simulink model "aBaja2026"  (R2026a)
settings: Solver=FixedStepAuto  StartTime=0  StopTime=1000  FixedStep=timeStep
PostLoadFcn:
  | helperSLTrajectoryFollowerWithRRScenarioSetup
InitFcn:
  | helperSLTrajectoryFollowerWithRRScenarioSetup
  | worldActor=rrSim.getScenario();
  | world = worldActor.actor_spec.world_spec;
  | % Inputs you already have (example):
  | EgoActorID  = 1;
  | egoSetSpeed = 0;
  | 
  | % Get world + actors
  | 
  | 
  | % --- Find the ego actor (vectorized, minimal overhead) ---
  | actorIDs = arrayfun(@(a) str2double(a.actor_runtime.id), world.actors);
  | idx = (actorIDs == EgoActorID);
  | 
  | if nnz(idx) ~= 1
  |     error("Actor with ActorID:%d does not exist (or is not unique).", EgoActorID);
  | end
  | 
  | ego = world.actors(idx);
  | 
  | % --- Build 4x4 pose matrix quickly ---
  | temp_m = ego.actor_runtime.pose.matrix;
  | pose = [temp_m.col0.x temp_m.col1.x temp_m.col2.x temp_m.col3.x; ...
  |         temp_m.col0.y temp_m.col1.y temp_m.col2.y temp_m.col3.y; ...
  |         temp_m.col0.z temp_m.col1.z temp_m.col2.z temp_m.col3.z; ...
  |         temp_m.col0.w temp_m.col1.w temp_m.col2.w temp_m.col3.w];
  | 
  | rotm = pose(1:3,1:3);
  | pos  = pose(1:3,4)';   % [x y z] meters
  | 
  | % --- Euler angles from rotation matrix (ZYX: yaw, pitch, roll) ---
  | % If you have Robotics System Toolbox, rotm2eul exists; otherwise keep internal.
  | if exist("rotm2eul","file")
  |     eulZYX = rotm2eul(rotm,"ZYX");                 % radians: [yaw pitch roll]
  | else
  |     eulZYX = robotics.internal.rotm2eul(rotm,"ZYX");% radians: [yaw pitch roll]
  | end
  | 
  | % RoadRunner yaw -> conventional yaw:
  | yawDeg   = rad2deg(eulZYX(1)) + 90;
  | yawDeg   = mod(yawDeg + 180, 360) - 180;           % wrap to (-180,180]
  | pitchDeg = rad2deg(eulZYX(2));
  | rollDeg  = rad2deg(eulZYX(3));
  | 
  | % --- (Optional) reproduce your actorPose struct (kept consistent) ---
  | vGlobal = [egoSetSpeed*cosd(yawDeg), egoSetSpeed*sind(yawDeg), 0];
  | vBody   = (rotm' * vGlobal')';                      % body-fixed velocity
  | 
  | actorPose = struct( ...
  |     'ActorID', double(EgoActorID), ...
  |     'Position', pos, ...
  |     'Velocity', vGlobal, ...
  |     'vehicleFrameVelocity', [vBody(2), -vBody(1), vBody(3)], ...
  |     'Roll',  rollDeg, ...
  |     'Pitch', pitchDeg, ...
  |     'Yaw',   yawDeg, ...
  |     'AngularVelocity', [0 0 0]);
  | 
  | % --- Inline replacement for poseToSim3DInputs ---
  | % IMPORTANT: your original poseToSim3DInputs uses radians (pi terms),
  | % but getActorPose produced degrees. Fix by converting degrees -> radians here.
  | rollRad  = deg2rad(rollDeg);
  | pitchRad = deg2rad(pitchDeg);
  | yawRad   = deg2rad(yawDeg);
  | 
  | initialPosition = pos.*[1 -1 1];                               % 1x3
  | initialRotation = [rollRad, pitchRad, - yawRad];
  | 
  | % (Optional) wrap sim3D yaw to [-pi, pi]
  | initialRotation(3) = mod(initialRotation(3) + pi, 2*pi) - pi;
  | 
  | % Your original outputs:
  | % [initialPosition, initialRotation] = poseToSim3DInputs(...)
undefined symbols (not defined in the file): Defined, Ego, Lane, LKA, m, matlabshared, n, Pose, Sim3dSensor, timeStep, User, Velocity
libraries: roadrunnerscenario x9, drivingvehiclecontroller x3, simulink_extras x3, sim3dautolib x2, drivingscenarioandsensors x1, sim3dcameralib x1, sim3dlib x1, simulink x1
(part 1 of 2)
CloseFcn:
  | helperSLTrajectoryFollowerWithRRScenarioCleanup
settings Model: Creator=The MathWorks, Inc.  LastModifiedBy=rithv
settings DataIOCC: InspectSignalLogs=on
settings RTWCC: GenCodeOnly=on  GenerateReport=on  TargetLang=C++
settings GRTTargetCC: TargetLangStandard=C++03 (ISO)  CodeInterfacePackaging=C++ class

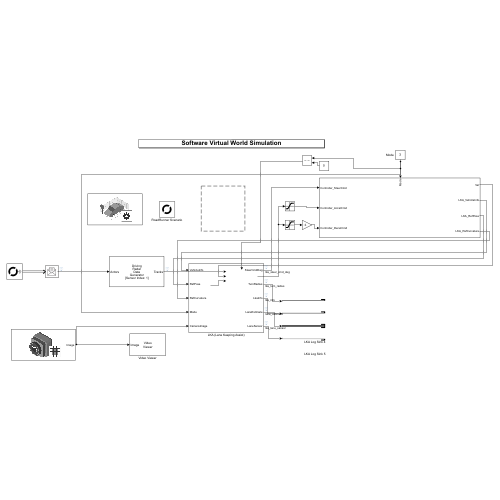
[thumbnail: Simulink's stored preview of the top-level diagram]
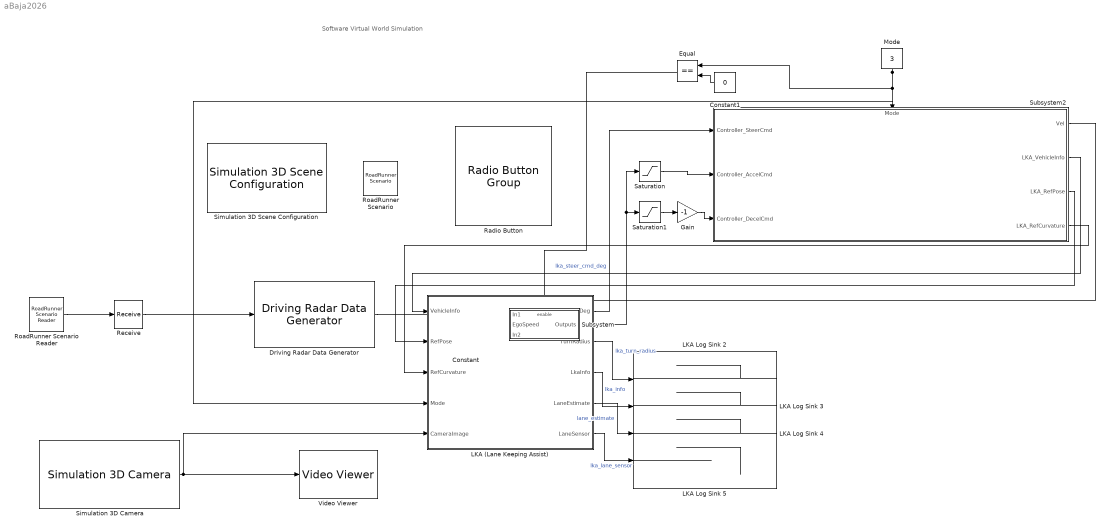
== system aBaja2026 ==
  note: Software Virtual World Simulation
  Constant : Constant  Value=8.3
  Constant1 : Constant  Value=0
  Driving Radar Data Generator : drivingscenarioandsensors/Driving Radar Data Generator  SensorIndex=1  UpdateRate=20  MountingLocation=[ 3.4, 0, 0.2 ]  MountingAngles=[0 0 0]  HasElevation=off  HasRangeRate=on  HasNoise=on  HasFalseAlarms=on  HasOcclusion=on  MaxNumReportsSource=Property  MaxNumReports=50  TargetReportFormat=Tracks  DetectionCoordinates=Body  TrackCoordinates=Body  BusNameSource=Auto  BusName=BusDrivingRadarDataGenerator  SimulateUsing=Interpreted execution  AzimuthResolution=4  ElevationResolution=5  RangeResolution=2.5  RangeRateResolution=0.5  AzimuthBiasFraction=0.1  ElevationBiasFraction=0.1  RangeBiasFraction=0.05  RangeRateBiasFraction=0.05  FieldOfView=[ 20, 5 ]  RangeLimits=[ 0, 150 ]  RangeRateLimits=[ -100, 100 ]  DetectionProbability=0.9  FalseAlarmRate=1e-06  ReferenceRange=100  ReferenceRCS=0  CenterFrequency=77e9  FilterInitializationFcn=initcvekf  ConfirmationThreshold=[2 3]  DeletionThreshold=[5 5]  InitialSeedSource=Repeatable  InitialSeed=0  UsedSeed=matlabshared.tracking.internal.SimulinkUtilities.seedManager(gcb)  ProfilesSource=From Scenario Reader block  ProfilesParameters=driving.internal.ActorProfilesRadarParameters  ProfilesExpression=struct('ClassID',0,'Length',4.7,'Width',1.8,'Height',1.4,'OriginOffset',[-1.35 0 0],'RCSPattern',[10 10;10 10],'RCSAzimuthAngles',[-180 180],'RCSElevationAngles',[-90 90])
  Equal : RelationalOperator  Operator===  OutDataTypeStr=boolean  RndMeth=Simplest  InputSameDT=off
  Gain : Gain  Gain=-1
  LKA (Lane Keeping Assist) : Subsystem  Description=aBaja 2026 LKA: lane source (camera detector YOLOP / team CNN / classic, or emulated for development), wheel-speed and gyro models, LKA_Controller (lane tracker, supervisor, pure pursuit / Stanley 2025 / MPC, a_y-jerk limiter, actuator manager). Output: road-wheel angle [deg, + left] to Subsystem2/Controller_SteerCmd.
  LKA Log Sink {2..5} (4 alike) : Terminator
  Mode : Constant  Value=3
  Radio Button : RadioButtonGroup  SelectedLabel=No Controller  ButtonGroupName=Event
  Receive : Receive  InputPortMessageModes=m  UseInternalQueue=off  QueueOverwriting=on  QueueLength=1  QueueType=LIFO
  RoadRunner Scenario : roadrunnerscenario/RoadRunner Scenario  ScenarioFileName=auto  ActorIDLinkedToModel=1  SampleTime=0.02  OpenRoadRunnerAtSimulationStart=on  EnableSimulationLoggingInRoadRunner=off  UserDefinedActions={}  UserDefinedEvents={}  PathPoints=500
  RoadRunner Scenario Reader : roadrunnerscenario/RoadRunner Scenario Reader  TopicCategory=Sensor  ActorCategory=All Types  ActionType=Path Following  EventType=User-Defined  TopicType=Actor Specifications  VehicleType=Vehicle Specifications  TrafficSignalType=Traffic Signal Specifications  TrafficSignalControllerType=Traffic Signal Controller Specifications  UserDefinedAction=Action1  UserDefinedEvent=Event1  Filter=Self  AdditionalRelationship=None  SensorTopic=Target Poses  LaneBoundaryOutputTopic=Ego-Lane  SensorID=1  SampleTime=0
  Saturation : Saturate  UpperLimit=2  LowerLimit=0
  Saturation1 : Saturate  UpperLimit=0  LowerLimit=-10
  Simulation 3D Camera : sim3dcameralib/Simulation 3D Camera  Priority=1  sensorTag=Sim3dSensor�  sensorId=1  sensorName=Sim3dSensor�  vehTagList={'Scene Origin';'SimulinkVehicle1';'SimulinkVehicle5'}  vehTag=SimulinkVehicle5  CoordinateSystem=ISO8855  mountLoc=Hood center  offsetFlag=off  tmountOffset=[0, 0, 0]  extTmount=off  rmountOffset=[0, 0, 0]  extRmount=off  FocalLength=[1109, 1109]  OpticalCenter=[640, 360]  ImageSize=[720, 1280]  RadialDistortion=[0, 0]  TangentialDistortion=[0, 0]  SensorSkew=0  VisualizeFieldOfView=on  FieldOfViewRange=61  DepthOutportEnabled=off  SemanticOutportEnabled=off  TransformOutportEnabled=off  SampleTime=-1  mountPoint=[0 0 0]  mountOrientation=[0 0 0]  aMode=3  ID=1
      settings: LibrarySourceBlock=drivingsim3d/Simulation 3D Camera
  Simulation 3D Scene Configuration : sim3dlib/Simulation 3D Scene Configuration  Priority=0  ProjectFormat=RoadRunner  SceneDesc=Straight road  ProjectName=D:\toolbox\shared\sim3d_projects\automotive_project_windows\UE\WindowsNoEditor\VehicleSimulation.exe  ScenePath=/Game/Maps/HwStrght  RoadRunnerProjectPath=D:\Work\25b\aBaja\SoftwareVirtualWorldSimulation\resources\UnrealFiles\AEB.usd  EnableOpenDRIVE=off  vehTagList={'Custom';'Scene Origin';'SimulinkVehicle1';'SimulinkVehicle5'}  vehTag=SimulinkVehicle5  AttachedCameraRelativeTranslation=[0 0 0]  FreeCameraDefaultInitialTranslation=[-6, 0, 2]  AttachedCameraRelativeRotation=[0 0 0]  FreeCameraDefaultInitialRotation=[0, -15, 0]  ViewpointName=Custom  FreeCameraInitialTranslation=[0 0 0]  FreeCameraInitialRotation=[0 0 0]  OpVisEn=off  Ts=timeStep  EnableWindow=off  EnableRemoteAccess=off  SimulationMode=CoSimulation  SimulateUsing=Interpreted execution  EnableAnimationRecording=off  OverrideDefaultRecording=off  AnimationRecordingFileName=sim3dAnimation.mat  AnimationRecordingInterval=[0 inf]  EnableWeather=off  SunAzimuth=90  SunAltitude=40.0  EnableGeospatialSun=off  Latitude=0  Longitude=0  Date=2023-01-01  Time=10:30:00  GeoTimeZone=-5.0  SunDaylightSaving=off  wind=1  clouds=10  EnableVolumetricClouds=off  CloudCoverage=0  CloudAltitude=6  fog=0  rain=0  RaindropsEffect=off  SnowDensity=0  EnableGeospatial=off  TilesetSource=Earth terrain  UseTrueOrigin=off  OriginHeight=200  OriginLatitude=40.744652  OriginLongitude=-73.988864  MapStyle=Aerial  AdditionalAssetIDs=[]  UseAdvancedSunSky=off  SolarTime=11  TimeZone=-5  Day=21  Month=9  Year=2022  UseDaylightSavingTime=on  DSTStartDay=10  DSTStartMonth=3  DSTEndDay=3  DSTEndMonth=11  DSTSwitchHour=2  sensorTag=MainCamera1  sensorId=1  sensorName=MainCamera1  mountLoc=Origin  offsetFlag=off  tmountOffset=[0, 0, 0]  rmountOffset=[0, 0, 0]  HorizontalResolution=1280  VerticalResolution=720  HorizontalFOV=60  mountPoint=[0 0 0]  mountOrientation=[0 0 0]  aMode=3  ID=1  GeoTrigger=Inactive  ViewNameList={'Custom'}  ViewTranslationList={'[0 0 0]'}  ViewRotationList={'[0 0 0]'}
      settings: LibrarySourceBlock=drivingsim3d/Simulation 3D Scene Configuration
  Subsystem : Subsystem
  Subsystem2 : Subsystem
      settings: PortSchema="{\"entries\":[{\"content\":{\"sides\":[{\"content\":{\"connectorIds\":[\"In1\",\"In2\",\"In3\"]},\"type\":\"ConnectorPlacement.EquallySpacedRectSide\",\"uuid\":\"2aff80b0-242f-49d2-ab36-0fd5582041a3\"},{\"content\":{\"connectorIds\":[\"Out1\",\"Out2\",\"Out3\",\"Out4\"],\"side\":\"RIGHT\"},\"type\":\"ConnectorPlacement.EquallySpacedRectSide\",\"uuid\":\"d3dd7aef-9728-4256-afed-548c516fba6e\"},{\"content\":{\"connectorIds\":[\"In4\"],\"side\":\"TOP\"},\"type\":\"ConnectorPlacement.EquallySpacedRectSide\",\"uuid\":\"fab05331-aabf-476e-ad1f-b5e3b7241bda\"}]},\"type\":\"ConnectorPlacement.EquallySpacedConnector\",\"uuid\":\"5fa4dbc3-4efd-4194-96c5-15d00eaf64f3\"}],\"packageUris\":[\"http://schema.mathworks.com/mf0/Connector/R2020b\"],\"version\":\"1.0\"}"
  Video Viewer : VideoViewer  FigPos=[1 1150 1920 1053]
  wires:
  RoadRunner Scenario Reader/1 -> Receive/1
  Receive/1 -> Driving Radar Data Generator/1
  Driving Radar Data Generator/1 -> Subsystem/1(In1)
  Subsystem2/1(Vel) -> Subsystem/2(EgoSpeed)
  Constant/1 -> Subsystem/3(In2)
  Subsystem/1(Outputs) -> Saturation/1, Saturation1/1
  Saturation/1 -> Subsystem2/2(Controller_AccelCmd)
  Saturation1/1 -> Gain/1
  Gain/1 -> Subsystem2/3(Controller_DecelCmd)
  Mode/1 -> Subsystem2/4(Mode), Equal/1, LKA (Lane Keeping Assist)/4(Mode)
  Equal/1 -> Subsystem/Enable
  Constant1/1 -> Equal/2
  Simulation 3D Camera/1 -> Video Viewer/1, LKA (Lane Keeping Assist)/5(CameraImage)
  Subsystem2/2(LKA_VehicleInfo) -> LKA (Lane Keeping Assist)/1(VehicleInfo)
  Subsystem2/3(LKA_RefPose) -> LKA (Lane Keeping Assist)/2(RefPose)
  Subsystem2/4(LKA_RefCurvature) -> LKA (Lane Keeping Assist)/3(RefCurvature)
  LKA (Lane Keeping Assist)/1(SteerCmdDeg) -> Subsystem2/1(Controller_SteerCmd)  "lka_steer_cmd_deg"
  LKA (Lane Keeping Assist)/2(TurnRadius) -> LKA Log Sink 2/1  "lka_turn_radius"
  LKA (Lane Keeping Assist)/3(LkaInfo) -> LKA Log Sink 3/1  "lka_info"
  LKA (Lane Keeping Assist)/4(LaneEstimate) -> LKA Log Sink 4/1  "lane_estimate"
  LKA (Lane Keeping Assist)/5(LaneSensor) -> LKA Log Sink 5/1  "lka_lane_sensor"

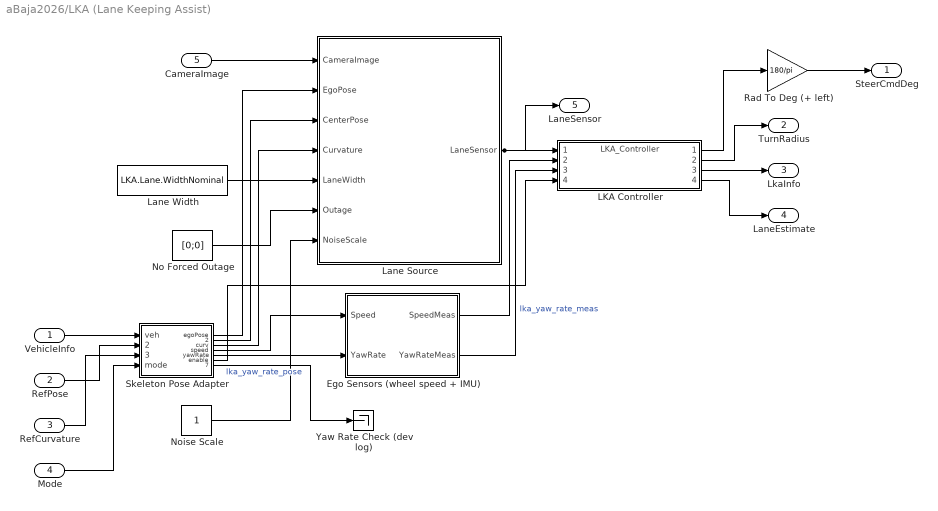
== system aBaja2026/LKA (Lane Keeping Assist) ==
  VehicleInfo : Inport
  RefPose : Inport  Port=2
  RefCurvature : Inport  Port=3
  Mode : Inport  Port=4
  CameraImage : Inport  Port=5
  Ego Sensors (wheel speed + IMU) : Subsystem
  LKA Controller : ModelReference  ModelNameDialog=LKA_Controller  SimulationMode=Normal  ModelReferenceVersion=1.1
  Lane Source : Subsystem  Variant=on
  Lane Width : Constant  Value=LKA.Lane.WidthNominal  SampleTime=LKA.Ts
  No Forced Outage : Constant  Value=[0;0]  SampleTime=LKA.Ts
  Noise Scale : Constant  SampleTime=LKA.Ts
  Rad To Deg (+ left) : Gain  Gain=180/pi
  Skeleton Pose Adapter : MATLAB Function  TreatAsAtomicUnit=on
  Yaw Rate Check (dev log) : Terminator
  SteerCmdDeg : Outport
  TurnRadius : Outport  Port=2
  LkaInfo : Outport  Port=3
  LaneEstimate : Outport  Port=4
  LaneSensor : Outport  Port=5
  wires:
  RefCurvature/1 -> Skeleton Pose Adapter/3(refCurv)
  VehicleInfo/1 -> Skeleton Pose Adapter/1(veh)
  No Forced Outage/1 -> Lane Source/6(Outage)
  LKA Controller/1 -> Rad To Deg (+ left)/1
  Lane Width/1 -> Lane Source/5(LaneWidth)
  RefPose/1 -> Skeleton Pose Adapter/2(refPose)
  Skeleton Pose Adapter/5(yawRate) -> Ego Sensors (wheel speed + IMU)/2(YawRate)
  Mode/1 -> Skeleton Pose Adapter/4(mode)
  CameraImage/1 -> Lane Source/1(CameraImage)
  Skeleton Pose Adapter/1(egoPose) -> Lane Source/2(EgoPose)
  Skeleton Pose Adapter/2(centerPose) -> Lane Source/3(CenterPose)
  Skeleton Pose Adapter/3(curv) -> Lane Source/4(Curvature)
  Skeleton Pose Adapter/4(speed) -> Ego Sensors (wheel speed + IMU)/1(Speed)
  LKA Controller/4 -> LaneEstimate/1
  Skeleton Pose Adapter/6(enable) -> LKA Controller/4
  Skeleton Pose Adapter/7(yawRatePose) -> Yaw Rate Check (dev log)/1  "lka_yaw_rate_pose"
  Ego Sensors (wheel speed + IMU)/1(SpeedMeas) -> LKA Controller/2
  Noise Scale/1 -> Lane Source/7(NoiseScale)
  Lane Source/1(LaneSensor) -> LaneSensor/1, LKA Controller/1
  Ego Sensors (wheel speed + IMU)/2(YawRateMeas) -> LKA Controller/3  "lka_yaw_rate_meas"
  LKA Controller/3 -> LkaInfo/1
  LKA Controller/2 -> TurnRadius/1
  Rad To Deg (+ left)/1 -> SteerCmdDeg/1

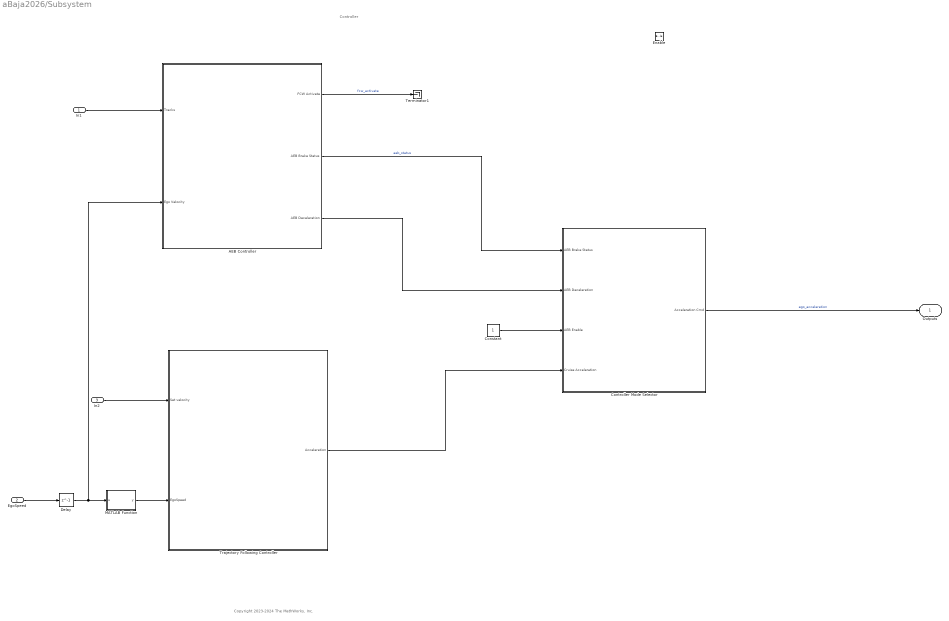
== system aBaja2026/Subsystem ==
  note: Controller
  note: Copyright 2023-2024 The MathWorks, Inc.
  In1 : Inport
  EgoSpeed : Inport  Port=2
  In2 : Inport  Port=3
  Enable : EnablePort
  AEB Controller : Subsystem
  Constant : Constant
  Controller Mode Selector : Subsystem
  Delay : Delay  DelayLength=1  InitialCondition=[0 0 0]
  MATLAB Function : MATLAB Function  TreatAsAtomicUnit=on
  Terminator1 : Terminator
  Trajectory Following Controller : Subsystem
  Outputs : Outport
  wires:
  Trajectory Following Controller/1(Acceleration) -> Controller Mode Selector/4(Cruise Acceleration)
  Delay/1 -> MATLAB Function/1(u), AEB Controller/2(Ego Velocity)
  In2/1 -> Trajectory Following Controller/1(Set velocity)
  MATLAB Function/1(y) -> Trajectory Following Controller/2(EgoSpeed)
  Controller Mode Selector/1(Acceleration Cmd) -> Outputs/1  "ego_acceleration"
  In1/1 -> AEB Controller/1(Tracks)
  AEB Controller/2(AEB Brake Status) -> Controller Mode Selector/1(AEB Brake Status)  "aeb_status"
  EgoSpeed/1 -> Delay/1
  Constant/1 -> Controller Mode Selector/3(AEB Enable)
  AEB Controller/1(FCW Activate) -> Terminator1/1  "fcw_activate"
  AEB Controller/3(AEB Deceleration) -> Controller Mode Selector/2(AEB Deceleration)

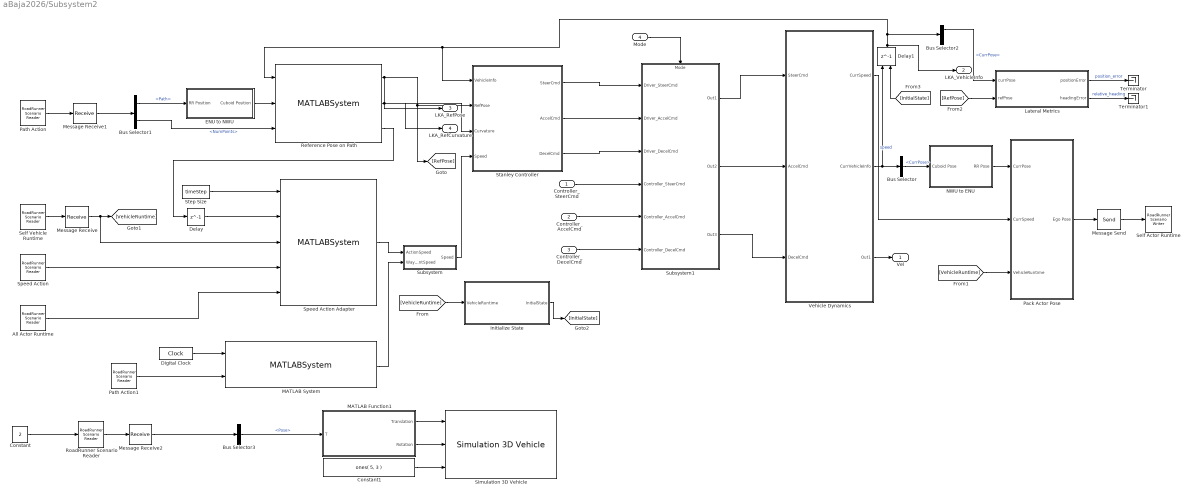
== system aBaja2026/Subsystem2 ==
  Controller_SteerCmd : Inport
  Controller_AccelCmd : Inport  Port=2
  Controller_DecelCmd : Inport  Port=3
  Mode : Inport  Port=4
  All Actor Runtime : roadrunnerscenario/RoadRunner Scenario Reader  TopicCategory=Actor  ActorCategory=All Types  ActionType=Path Following  EventType=User-Defined  TopicType=Actor Pose  VehicleType=Vehicle Specifications  TrafficSignalType=Traffic Signal Specifications  TrafficSignalControllerType=Traffic Signal Controller Specifications  UserDefinedAction=Action1  UserDefinedEvent=Event1  Filter=None  AdditionalRelationship=None  SensorTopic=Target Poses  LaneBoundaryOutputTopic=Ego-Lane  SensorID=1  SampleTime=0
  Bus Selector : BusSelector  OutputSignals=CurrPose
  Bus Selector1 : BusSelector  OutputSignals=PathTarget.Path,PathTarget.NumPoints
  Bus Selector2 : BusSelector  OutputSignals=CurrPose,CurrVelocity
  Bus Selector3 : BusSelector  OutputSignals=ActorRuntime.Pose
  Constant : Constant  Value=2  OutDataTypeStr=uint64
  Constant1 : Constant  Value=ones( 5, 3 )
  Delay : Delay  DelayLength=1  InitialCondition=logical(0)
  Delay1 : Delay  DelayLength=1  InitialConditionSource=Input port
      settings: InputPortMap=u0,p4
  Digital Clock : DigitalClock  SampleTime=-1
  ENU to NWU : Subsystem
  Initialize State : Subsystem
  Lateral Metrics : MATLAB Function  TreatAsAtomicUnit=on
  MATLAB Function1 : MATLAB Function  TreatAsAtomicUnit=on
  MATLAB System : MATLABSystem  InputPortMessageModes=n,m  System=getEgoSpeed  MaxNumPoints=5000
      mask Type: getEgoSpeed
  Message Receive : Receive  InputPortMessageModes=m
  Message Receive1 : Receive  InputPortMessageModes=m
  Message Receive2 : Receive  InputPortMessageModes=m
  Message Send : Send  OutputPortMessageModes=m
  NWU to ENU : Subsystem
  Pack Actor Pose : Subsystem
  Path Action : roadrunnerscenario/RoadRunner Scenario Reader  TopicCategory=Action  ActorCategory=All Types  ActionType=Path Following  EventType=User-Defined  TopicType=Actor Specifications  VehicleType=Vehicle Specifications  TrafficSignalType=Traffic Signal Specifications  TrafficSignalControllerType=Traffic Signal Controller Specifications  UserDefinedAction=Action1  UserDefinedEvent=Event1  Filter=Self  AdditionalRelationship=None  SensorTopic=Target Poses  LaneBoundaryOutputTopic=Ego-Lane  SensorID=1  SampleTime=0
  Path Action1 : roadrunnerscenario/RoadRunner Scenario Reader  TopicCategory=Action  ActorCategory=All Types  ActionType=Path Following  EventType=User-Defined  TopicType=Actor Specifications  VehicleType=Vehicle Specifications  TrafficSignalType=Traffic Signal Specifications  TrafficSignalControllerType=Traffic Signal Controller Specifications  UserDefinedAction=Action1  UserDefinedEvent=Event1  Filter=Self  AdditionalRelationship=None  SensorTopic=Target Poses  LaneBoundaryOutputTopic=Ego-Lane  SensorID=1  SampleTime=0
  Reference Pose on Path : MATLABSystem  System=HelperReferencePoseOnPath
      mask Type: HelperReferencePoseOnPath
  RoadRunner Scenario Reader : roadrunnerscenario/RoadRunner Scenario Reader  TopicCategory=Actor  ActorCategory=Vehicle  ActionType=Path Following  EventType=User-Defined  TopicType=Actor Specifications  VehicleType=Vehicle Pose  TrafficSignalType=Traffic Signal Specifications  TrafficSignalControllerType=Traffic Signal Controller Specifications  UserDefinedAction=Action1  UserDefinedEvent=Event1  Filter=Actor ID (provided by input)  AdditionalRelationship=None  SensorTopic=Target Poses  LaneBoundaryOutputTopic=Ego-Lane  SensorID=1  SampleTime=0
  Self Actor Runtime : roadrunnerscenario/RoadRunner Scenario Writer  TopicCategory=Actor  ActorCategory=All Types  EventType=Action Complete  UserDefinedEvent=Event1  VehicleType=Vehicle Pose  TopicType=Actor Pose
  Self Vehicle Runtime : roadrunnerscenario/RoadRunner Scenario Reader  TopicCategory=Actor  ActorCategory=Vehicle  ActionType=Path Following  EventType=User-Defined  TopicType=Actor Specifications  VehicleType=Vehicle Pose  TrafficSignalType=Traffic Signal Specifications  TrafficSignalControllerType=Traffic Signal Controller Specifications  UserDefinedAction=Action1  UserDefinedEvent=Event1  Filter=Self  AdditionalRelationship=None  SensorTopic=Target Poses  LaneBoundaryOutputTopic=Ego-Lane  SensorID=1  SampleTime=0
  Simulation 3D Vehicle : sim3dautolib/Simulation 3D Vehicle  Priority=-1  PassVehMesh=Muscle car  MeshPath=/MathWorksAutomotiveContent/Vehicles/Muscle/Meshes/SK_MuscleCar.SK_MuscleCar  VehColor=Black  ActorName=SimulinkVehicle1  VehLightsControl=off  HeadlightColor=[ 1, 1, 1 ]  HighBeamIntensity=100000  LowBeamIntensity=60000  HighBeamConeAngle=1.22  LowBeamConeAngle=1.22  LeftHeadlightOrientation=[ 0, 0 ]  RightHeadlightOrientation=[ 0, 0 ]  BrakelightIntensity=500  ReverselightIntensity=500  SignallightIntensity=500  SignallightPeriod=1  SignalPulseWidth=50  Translation=zeros( 5, 3 )  Rotation=zeros( 5, 3 )  Scale=ones( 5, 3 )  SampleTime=-1  ActorType=SimulinkVehicle  ID=1  aMode=2  ActorTag=SimulinkVehicle1
      settings: LibrarySourceBlock=vehdynlibsim3d/Simulation 3D Vehicle
  Speed Action : roadrunnerscenario/RoadRunner Scenario Reader  TopicCategory=Action  ActorCategory=All Types  ActionType=Speed Change  EventType=User-Defined  TopicType=Actor Specifications  VehicleType=Vehicle Specifications  TrafficSignalType=Traffic Signal Specifications  TrafficSignalControllerType=Traffic Signal Controller Specifications  UserDefinedAction=Action1  UserDefinedEvent=Event1  Filter=Self  AdditionalRelationship=None  SensorTopic=Target Poses  LaneBoundaryOutputTopic=Ego-Lane  SensorID=1  SampleTime=0
  Speed Action Adapter : MATLABSystem  InputPortMessageModes=n,n,n,m,m  System=HelperSpeedActionAdapter
      mask Type: HelperSpeedActionAdapter
  Stanley Controller : Subsystem
  Step Size : Constant  Value=timeStep
  Subsystem : Subsystem
  Subsystem1 : Subsystem
      settings: PortSchema="{\"entries\":[{\"content\":{\"sides\":[{\"content\":{\"connectorIds\":[\"In1\",\"In2\",\"In3\",\"In4\",\"In5\",\"In6\"]},\"type\":\"ConnectorPlacement.EquallySpacedRectSide\",\"uuid\":\"5e8a80cd-bbf2-4820-bc9c-ca402fa19997\"},{\"content\":{\"connectorIds\":[\"Out1\",\"Out2\",\"Out3\"],\"side\":\"RIGHT\"},\"type\":\"ConnectorPlacement.EquallySpacedRectSide\",\"uuid\":\"8f6bc7c9-4314-479c-a597-9e5289dcb804\"},{\"content\":{\"connectorIds\":[\"In7\"],\"side\":\"TOP\"},\"type\":\"ConnectorPlacement.EquallySpacedRectSide\",\"uuid\":\"02742dae-bcc0-42b0-9839-7c168f2ffa67\"}]},\"type\":\"ConnectorPlacement.EquallySpacedConnector\",\"uuid\":\"da407c9a-da98-4b96-8771-1dc16b41106f\"}],\"packageUris\":[\"http://schema.mathworks.com/mf0/Connector/R2020b\"],\"version\":\"1.0\"}"
  Terminator : Terminator
  Terminator1 : Terminator
  Vehicle Dynamics : Subsystem
  Vel : Outport
  LKA_VehicleInfo : Outport  Port=2
  LKA_RefPose : Outport  Port=3
  LKA_RefCurvature : Outport  Port=4
  wires:
  Message Send/1 -> Self Actor Runtime/1
  Constant/1 -> RoadRunner Scenario Reader/1
  Bus Selector3/1 -> MATLAB Function1/1(T)  "<Pose>"
  Self Vehicle Runtime/1 -> Message Receive/1
  Reference Pose on Path/1 -> [RefPose], Stanley Controller/2(RefPose), LKA_RefPose/1
  Step Size/1 -> Speed Action Adapter/1
  Message Receive/1 -> Speed Action Adapter/3, [VehicleRuntime]
  Controller_AccelCmd/1 -> Subsystem1/5(Controller_AccelCmd)
  Initialize State/1(InitialState) -> [InitialState]
  Controller_SteerCmd/1 -> Subsystem1/4(Controller_SteerCmd)
  Bus Selector/1 -> NWU to ENU/1(Cuboid Pose)  "<CurrPose>"
  Subsystem/1(Speed) -> Stanley Controller/4(Speed)
  [VehicleRuntime] -> Pack Actor Pose/3(VehicleRuntime)
  Subsystem1/2(Out2) -> Vehicle Dynamics/2(AccelCmd)
  Path Action1/1 -> MATLAB System/2
  MATLAB Function1/1(Translation) -> Simulation 3D Vehicle/1
  Delay/1 -> Speed Action Adapter/2
  Vehicle Dynamics/1(CurrSpeed) -> Pack Actor Pose/2(CurrSpeed)  "speed"
  [VehicleRuntime] -> Initialize State/1(VehicleRuntime)
  Pack Actor Pose/1(Ego Pose) -> Message Send/1
  Lateral Metrics/1(positionError) -> Terminator/1  "position_error"
  Subsystem1/3(Out3) -> Vehicle Dynamics/3(DecelCmd)
  Reference Pose on Path/3 -> Delay/1
  RoadRunner Scenario Reader/1 -> Message Receive2/1
  Message Receive2/1 -> Bus Selector3/1
  Vehicle Dynamics/2(CurrVehicleInfo) -> Bus Selector/1, Delay1/1
  Bus Selector1/2 -> Reference Pose on Path/3  "<NumPoints>"
  Message Receive1/1 -> Bus Selector1/1
  Reference Pose on Path/2 -> Stanley Controller/3(Curvature), LKA_RefCurvature/1
  [InitialState] -> Delay1/2
  Lateral Metrics/2(headingError) -> Terminator1/1  "relative_heading"
  ENU to NWU/1(Cuboid Position) -> Reference Pose on Path/2
  Delay1/1 -> Stanley Controller/1(VehicleInfo), Reference Pose on Path/1, Bus Selector2/1, LKA_VehicleInfo/1
  Stanley Controller/3(DecelCmd) -> Subsystem1/3(Driver_DecelCmd)
  All Actor Runtime/1 -> Speed Action Adapter/5
  Stanley Controller/2(AccelCmd) -> Subsystem1/2(Driver_AccelCmd)
  Bus Selector1/1 -> ENU to NWU/1(RR Position)  "<Path>"
  Path Action/1 -> Message Receive1/1
  Constant1/1 -> Simulation 3D Vehicle/3
  Digital Clock/1 -> MATLAB System/1
  Mode/1 -> Subsystem1/7(Mode)
  [RefPose] -> Lateral Metrics/2(refPose)
  Bus Selector2/1 -> Lateral Metrics/1(currPose)  "<CurrPose>"
  MATLAB Function1/2(Rotation) -> Simulation 3D Vehicle/2
  Speed Action/1 -> Speed Action Adapter/4
  Speed Action Adapter/1 -> Subsystem/1(ActionSpeed)
  MATLAB System/1 -> Subsystem/2(WayPointSpeed)
  Stanley Controller/1(SteerCmd) -> Subsystem1/1(Driver_SteerCmd)
  NWU to ENU/1(RR Pose) -> Pack Actor Pose/1(CurrPose)
  Controller_DecelCmd/1 -> Subsystem1/6(Controller_DecelCmd)
  Subsystem1/1(Out1) -> Vehicle Dynamics/1(SteerCmd)
  Vehicle Dynamics/3(Out1) -> Vel/1

== system aBaja2026/LKA (Lane Keeping Assist)/Ego Sensors (wheel speed + IMU) ==
  Speed : Inport
  YawRate : Inport  Port=2
  Gyro Noise : RandomNumber  Seed=LKA.EgoSen.Seed(2)  SampleTime=LKA.Ts
  Noise : Mux  Inputs=2
  Sensor Model : MATLAB Function  TreatAsAtomicUnit=on
  Speed Noise : RandomNumber  Seed=LKA.EgoSen.Seed(1)  SampleTime=LKA.Ts
  SpeedMeas : Outport
  YawRateMeas : Outport  Port=2
  wires:
  Speed/1 -> Sensor Model/1(v)
  YawRate/1 -> Sensor Model/2(r)
  Speed Noise/1 -> Noise/1
  Gyro Noise/1 -> Noise/2
  Noise/1 -> Sensor Model/3(n)
  Sensor Model/1(vMeas) -> SpeedMeas/1
  Sensor Model/2(rMeas) -> YawRateMeas/1

== system aBaja2026/LKA (Lane Keeping Assist)/Lane Source ==
  note: 1) Add Subsystem or Model blocks as valid variant choices.
      | 2) You cannot connect blocks at this level. At simulation, connectivity is automatically
      | determined, based on the active variant and port name matching.
  CameraImage : Inport
  EgoPose : Inport  Port=2
  CenterPose : Inport  Port=3
  Curvature : Inport  Port=4
  LaneWidth : Inport  Port=5
  Outage : Inport  Port=6
  NoiseScale : Inport  Port=7
  Camera Lane Detector : Subsystem  VariantControl=LKA_LANE_SOURCE == 1
  Emulated Lane Sensor (development only) : Subsystem  VariantControl=LKA_LANE_SOURCE == 2
  LaneSensor : Outport

== system aBaja2026/Subsystem/AEB Controller ==
  note: AEB Controller
  Tracks : Inport  SampleTime=timeStep  BusOutputAsStruct=on
  Ego Velocity : Inport  Port=2  PortDimensions=[1 3]
  Constant : Constant  Value=3.5
  Ego Speed : MATLAB Function  TreatAsAtomicUnit=on
  Emergency Braking Controller : Subsystem
  Find MIO : MATLAB Function  TreatAsAtomicUnit=on
  Position Selector : Constant  Value=|
      | [1 0 0 0 0 0;
      |                     0 1 0 0 0 0];
  FCW Activate : Outport  OutDataTypeStr=uint8  PortDimensions=1  VectorParamsAs1DForOutWhenUnconnected=off
  AEB Brake Status : Outport  Port=2  OutDataTypeStr=uint8  PortDimensions=1  VectorParamsAs1DForOutWhenUnconnected=off
  AEB Deceleration : Outport  Port=3
  wires:
  Find MIO/2(vx) -> Emergency Braking Controller/2(MIO Velocity)
  Position Selector/1 -> Find MIO/2(positionSelector)
  Ego Velocity/1 -> Ego Speed/1(velocity)
  Emergency Braking Controller/1(FCW Activate) -> FCW Activate/1  "fcw_activate"
  Emergency Braking Controller/3(Deceleration) -> AEB Deceleration/1
  Ego Speed/1(speed) -> Find MIO/4(egoSpeed), Emergency Braking Controller/4(Longitudinal Velocity)  "ego_velocity"
  Find MIO/1(x) -> Emergency Braking Controller/1(MIO Distance)
  Constant/1 -> Find MIO/3(laneWidth)
  Emergency Braking Controller/2(AEB Status) -> AEB Brake Status/1  "aeb_status"
  Find MIO/3(relativeYawAngle) -> Emergency Braking Controller/3(relativeYawAngle)
  Tracks/1 -> Find MIO/1(confirmedTracks)

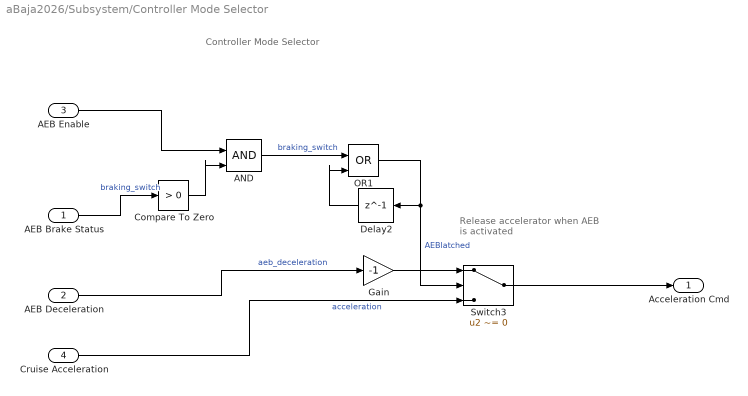
== system aBaja2026/Subsystem/Controller Mode Selector ==
  note: Release accelerator when AEB is activated
  note: Controller Mode Selector
  AEB Brake Status : Inport
  AEB Deceleration : Inport  Port=2
  AEB Enable : Inport  Port=3
  Cruise Acceleration : Inport  Port=4
  AND : Logic  IconShape=distinctive  AllPortsSameDT=off  OutDataTypeStr=boolean
  Compare To Zero : simulink/Logic and Bit Operations/Compare To Zero  relop=>  OutDataTypeStr=boolean
  Delay2 : Delay  DelayLength=1
  Gain : Gain  Gain=-1
  OR1 : Logic  Operator=OR  IconShape=distinctive  AllPortsSameDT=off  OutDataTypeStr=boolean
  Switch3 : Switch  Criteria=u2 ~= 0  SaturateOnIntegerOverflow=off  InputSameDT=off
  Acceleration Cmd : Outport
  wires:
  AND/1 -> OR1/1  "braking_switch"
  AEB Deceleration/1 -> Gain/1  "aeb_deceleration"
  Switch3/1 -> Acceleration Cmd/1
  Delay2/1 -> OR1/2
  Gain/1 -> Switch3/1
  OR1/1 -> Delay2/1, Switch3/2  "AEBlatched"
  Cruise Acceleration/1 -> Switch3/3  "acceleration"
  AEB Brake Status/1 -> Compare To Zero/1  "braking_switch"
  AEB Enable/1 -> AND/1
  Compare To Zero/1 -> AND/2

== system aBaja2026/Subsystem/Trajectory Following Controller ==
  note: Trajectory Following Controller
  Set velocity : Inport  SampleTime=timeStep
  EgoSpeed : Inport  Port=2
  Constant : Constant  SampleTime=timeStep
  Constant1 : Constant  Value=0
  Longitudinal Controller Stanley : drivingvehiclecontroller/Longitudinal Controller Stanley  Kp=2.5  Ki=1  SampleTime=timeStep  MaxAcceleration=2  MaxDeceleration=10
  Subtract : Sum  Inputs=+-
  Acceleration : Outport
  wires:
  Subtract/1 -> Acceleration/1
  Constant/1 -> Longitudinal Controller Stanley/3
  Constant1/1 -> Longitudinal Controller Stanley/4
  Longitudinal Controller Stanley/2 -> Subtract/2
  Longitudinal Controller Stanley/1 -> Subtract/1
  Set velocity/1 -> Longitudinal Controller Stanley/1
  EgoSpeed/1 -> Longitudinal Controller Stanley/2

== system aBaja2026/Subsystem2/ENU to NWU ==
  RR Position : Inport
  Gain : Gain  Gain=-1
  Matrix Concatenate : Concatenate  NumInputs=3  Mode=Multidimensional array  ConcatenateDimension=2
  Selector : Selector  NumberOfDimensions=2  InputPortWidth=3  IndexOptions=Select all,Index vector (dialog)  Indices=[1 3],1  OutputSizes=1,1
  Selector1 : Selector  NumberOfDimensions=2  InputPortWidth=3  IndexOptions=Select all,Index vector (dialog)  Indices=[1 3],2  OutputSizes=1,1
  Selector2 : Selector  NumberOfDimensions=2  InputPortWidth=3  IndexOptions=Select all,Index vector (dialog)  Indices=[1 3],3  OutputSizes=1,1
  Cuboid Position : Outport
  wires:
  Gain/1 -> Matrix Concatenate/2
  Selector1/1 -> Matrix Concatenate/1
  Selector2/1 -> Matrix Concatenate/3
  Selector/1 -> Gain/1
  RR Position/1 -> Selector/1, Selector1/1, Selector2/1
  Matrix Concatenate/1 -> Cuboid Position/1

== system aBaja2026/Subsystem2/Initialize State ==
  VehicleRuntime : Inport
  Calculate Initial States : Subsystem
  Constant : Constant  Value=0
  Delay : Delay  DelayLength=1  InitialCondition=1
  InitialState : Outport
  wires:
  Delay/1 -> Calculate Initial States/Trigger
  Constant/1 -> Delay/1
  Calculate Initial States/1(EgoInitialState) -> InitialState/1
  VehicleRuntime/1 -> Calculate Initial States/1(EgoRuntime)

== system aBaja2026/Subsystem2/NWU to ENU ==
  Cuboid Pose : Inport
  Gain1 : Gain  Gain=-1
  Matrix Concatenate : Concatenate  NumInputs=3  Mode=Multidimensional array  ConcatenateDimension=2
  Selector : Selector  InputPortWidth=3  IndexOptions=Index vector (dialog)  Indices=3  OutputSizes=1
  Selector1 : Selector  InputPortWidth=3  IndexOptions=Index vector (dialog)  Indices=1  OutputSizes=1
  Selector2 : Selector  InputPortWidth=3  IndexOptions=Index vector (dialog)  Indices=2  OutputSizes=1
  RR Pose : Outport
  wires:
  Matrix Concatenate/1 -> RR Pose/1
  Selector2/1 -> Gain1/1
  Selector1/1 -> Matrix Concatenate/2
  Selector/1 -> Matrix Concatenate/3
  Cuboid Pose/1 -> Selector1/1, Selector/1, Selector2/1
  Gain1/1 -> Matrix Concatenate/1

== system aBaja2026/Subsystem2/Pack Actor Pose ==
  CurrPose : Inport
  CurrSpeed : Inport  Port=2
  VehicleRuntime : Inport  Port=3
  Assign : BusAssignment  AssignedSignals=Pose,Velocity
  Bus Selector : BusSelector  OutputSignals=ActorRuntime
  Pose Generation : MATLAB Function  TreatAsAtomicUnit=on
  Selector : Selector  InputPortWidth=3  IndexOptions=Index vector (dialog)  Indices=3  OutputSizes=1
  Velocity XYZ Components : MATLAB Function  TreatAsAtomicUnit=on
  Ego Pose : Outport
  wires:
  Velocity XYZ Components/1(velocity) -> Assign/3  "Velocity"
  Pose Generation/1(currPose) -> Assign/2  "Pose"
  CurrPose/1 -> Selector/1, Pose Generation/1(pose)
  Selector/1 -> Velocity XYZ Components/1(yaw)
  CurrSpeed/1 -> Velocity XYZ Components/2(speed)
  VehicleRuntime/1 -> Bus Selector/1
  Bus Selector/1 -> Assign/1  "<ActorRuntime>"
  Assign/1 -> Ego Pose/1

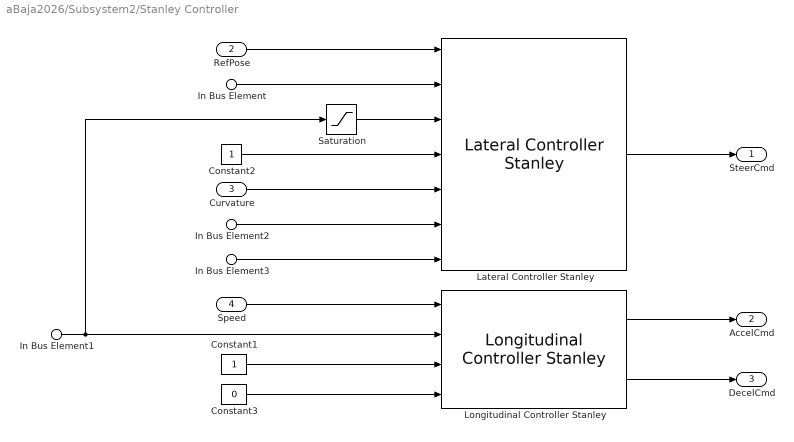
== system aBaja2026/Subsystem2/Stanley Controller ==
  In Bus Element : Inport  PortName=VehicleInfo  Element=CurrPose
  In Bus Element1 : Inport  PortName=VehicleInfo  Element=CurrVelocity
  In Bus Element2 : Inport  PortName=VehicleInfo  Element=CurrYawRate
  In Bus Element3 : Inport  PortName=VehicleInfo  Element=CurrSteer
  RefPose : Inport  Port=2
  Curvature : Inport  Port=3
  Speed : Inport  Port=4
  Constant1 : Constant
  Constant2 : Constant
  Constant3 : Constant  Value=0
  Lateral Controller Stanley : drivingvehiclecontroller/Lateral Controller Stanley  ModelType=Dynamic bicycle model  PositionGainF=3  PositionGainR=2.5  YawRateGain=0.2  DelayGain=0.2  VehicleMass=m  Lf=lf  Lr=lr  TireStiffness=70e3  Wheelbase=2.8  MaxSteeringAngle=90
  Longitudinal Controller Stanley : drivingvehiclecontroller/Longitudinal Controller Stanley  Kp=1  Ki=1  SampleTime=timeStep  MaxAcceleration=max_ac  MaxDeceleration=max_dc
  Saturation : Saturate  UpperLimit=inf  LowerLimit=0
  SteerCmd : Outport
  AccelCmd : Outport  Port=2
  DecelCmd : Outport  Port=3
  wires:
  In Bus Element/1 -> Lateral Controller Stanley/2
  Lateral Controller Stanley/1 -> SteerCmd/1
  In Bus Element2/1 -> Lateral Controller Stanley/6
  In Bus Element1/1 -> Saturation/1, Longitudinal Controller Stanley/2
  Constant1/1 -> Longitudinal Controller Stanley/3
  Longitudinal Controller Stanley/2 -> DecelCmd/1
  Constant2/1 -> Lateral Controller Stanley/4
  In Bus Element3/1 -> Lateral Controller Stanley/7
  Constant3/1 -> Longitudinal Controller Stanley/4
  RefPose/1 -> Lateral Controller Stanley/1
  Longitudinal Controller Stanley/1 -> AccelCmd/1
  Curvature/1 -> Lateral Controller Stanley/5
  Speed/1 -> Longitudinal Controller Stanley/1
  Saturation/1 -> Lateral Controller Stanley/3

== system aBaja2026/Subsystem2/Subsystem ==
  ActionSpeed : Inport
  WayPointSpeed : Inport  Port=2
  Switch : Switch  Criteria=u2 > Threshold  SaturateOnIntegerOverflow=off  InputSameDT=off
  Speed : Outport
  wires:
  ActionSpeed/1 -> Switch/1, Switch/2
  WayPointSpeed/1 -> Switch/3
  Switch/1 -> Speed/1

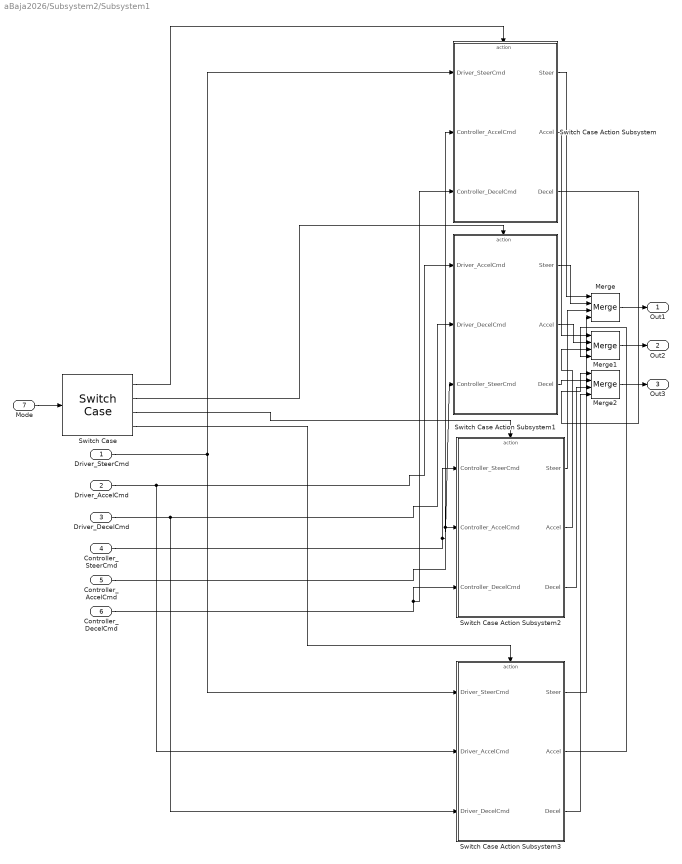
== system aBaja2026/Subsystem2/Subsystem1 ==
  Driver_SteerCmd : Inport
  Driver_AccelCmd : Inport  Port=2
  Driver_DecelCmd : Inport  Port=3
  Controller_SteerCmd : Inport  Port=4
  Controller_AccelCmd : Inport  Port=5
  Controller_DecelCmd : Inport  Port=6
  Mode : Inport  Port=7
  Merge : Merge  Inputs=4
  Merge1 : Merge  Inputs=4
  Merge2 : Merge  Inputs=4
  Switch Case : SwitchCase  CaseConditions={0,1,2,3}  ShowDefaultCase=off
  Switch Case Action Subsystem : Subsystem  TreatAsAtomicUnit=on
  Switch Case Action Subsystem1 : Subsystem  TreatAsAtomicUnit=on
  Switch Case Action Subsystem2 : Subsystem  TreatAsAtomicUnit=on
  Switch Case Action Subsystem3 : Subsystem  TreatAsAtomicUnit=on
  Out1 : Outport
  Out2 : Outport  Port=2
  Out3 : Outport  Port=3
  wires:
  Mode/1 -> Switch Case/1
  Controller_SteerCmd/1 -> Switch Case Action Subsystem1/3(Controller_SteerCmd), Switch Case Action Subsystem2/1(Controller_SteerCmd)
  Merge/1 -> Out1/1
  Switch Case/1 -> Switch Case Action Subsystem/Action
  Driver_DecelCmd/1 -> Switch Case Action Subsystem3/3(Driver_DecelCmd), Switch Case Action Subsystem1/2(Driver_DecelCmd)
  Switch Case/2 -> Switch Case Action Subsystem1/Action
  Switch Case/3 -> Switch Case Action Subsystem2/Action
  Merge1/1 -> Out2/1
  Driver_AccelCmd/1 -> Switch Case Action Subsystem3/2(Driver_AccelCmd), Switch Case Action Subsystem1/1(Driver_AccelCmd)
  Driver_SteerCmd/1 -> Switch Case Action Subsystem3/1(Driver_SteerCmd), Switch Case Action Subsystem/1(Driver_SteerCmd)
  Controller_AccelCmd/1 -> Switch Case Action Subsystem/2(Controller_AccelCmd), Switch Case Action Subsystem2/2(Controller_AccelCmd)
  Controller_DecelCmd/1 -> Switch Case Action Subsystem/3(Controller_DecelCmd), Switch Case Action Subsystem2/3(Controller_DecelCmd)
  Switch Case Action Subsystem/1(Steer) -> Merge/1
  Switch Case Action Subsystem/2(Accel) -> Merge1/1
  Switch Case Action Subsystem2/3(Decel) -> Merge2/3
  Switch Case Action Subsystem/3(Decel) -> Merge2/1
  Switch Case Action Subsystem1/1(Steer) -> Merge/2
  Switch Case Action Subsystem1/2(Accel) -> Merge1/2
  Switch Case Action Subsystem1/3(Decel) -> Merge2/2
  Switch Case Action Subsystem2/1(Steer) -> Merge/3
  Switch Case Action Subsystem2/2(Accel) -> Merge1/3
  Merge2/1 -> Out3/1
  Switch Case Action Subsystem3/1(Steer) -> Merge/4
  Switch Case Action Subsystem3/2(Accel) -> Merge1/4
  Switch Case Action Subsystem3/3(Decel) -> Merge2/4
  Switch Case/4 -> Switch Case Action Subsystem3/Action

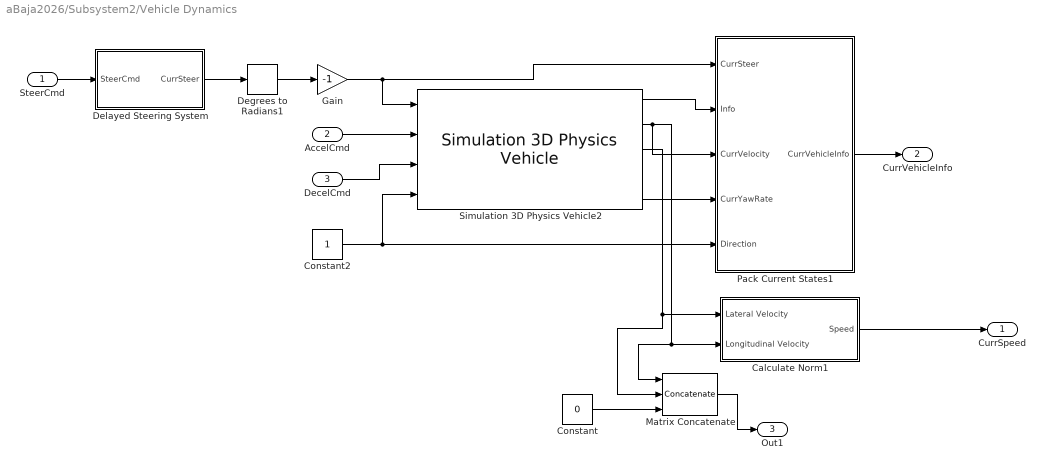
== system aBaja2026/Subsystem2/Vehicle Dynamics ==
  SteerCmd : Inport
  AccelCmd : Inport  Port=2
  DecelCmd : Inport  Port=3
  Calculate Norm1 : Subsystem
  Constant : Constant  Value=0
  Constant2 : Constant
  Degrees to Radians1 : simulink_extras/Transformations/Degrees to Radians
  Delayed Steering System : Subsystem
  Gain : Gain  Gain=-1
  Matrix Concatenate : Concatenate  NumInputs=3  Mode=Multidimensional array  ConcatenateDimension=2
  Pack Current States1 : Subsystem
  Simulation 3D Physics Vehicle2 : sim3dautolib/Simulation 3D Physics Vehicle  PassVehMesh=Muscle car  VehColor=Red  ActorName=SimulinkVehicle5  MeshPath=/MathWorksSimulation/Vehicles/Muscle/Meshes/SK_MuscleCar.SK_Sedan  TrackWidth=2  WheelBase=3  FrntWhlRadius=0.30  RearWhlRadius=0.30  FrntWhlWidth=0.20  RearWhlWidth=0.20  InitialPos=initialPosition  InitialRot=initialRotation  Mass=1500  CgOffset=[ 0, 0, 0 ]  IvehScale=[ 1, 1, 1 ]  ChassisHeight=1.5  Cd=0.3  Cl=0.1  TrqCrv=[75, 300, 400, 0 ]  SpdCrv=[ 0, 1000, 5500, 8000 ]  MaxRPM=10000  Jmot=1  bEngMax=0.15  bEngMin=2  DrivetrainType=Rear Wheel Drive  FrontRearSplit=0.5  TransType=Automatic  G=[-1 0 1 2 3 4 5 6 7 8]  N=[ -3.5 1 4.75 3.75 3.25 2.75 2.25 1.5 1 0.75]  UpShiftRPM=4000  DownShiftRPM=2000  MinRPM=750  tShift=.1  NDiff=3.2  eta=0.94  SteerType=Ackermann  SteerAngleRatio=1.0  EnableFrontSteer=on  FrntWhlMaxSteer=deg2rad(90)  EnableRearSteer=off  RearWhlMaxSteer=0  SteerSpdFctTbl=[ 1, 0.8, 0.7 ]  SteerVehSpdBpts=[ 0, 60, 120 ]./3.6  FrntWhlMaxTrq=1500  RearWhlMaxTrq=1500  HndBrkEnable=off  FrntWhlHndBrkEnable=off  RearWhlHndBrkEnable=off  FrntWhlMaxHndBrkTrq=3000  RearWhlMaxHndBrkTrq=1500  FrntSuspFOffset=[0 0 0]  RearSuspFOffset=[0 0 0]  FrntSuspMaxComp=0.15  RearSuspMaxComp=0.15  FrntSpringPreload=200  RearSpringPreload=200  FrntSpringRate=30e3  RearSpringRate=30e3  FrntSuspMaxExt=0.1  RearSuspMaxExt=0.1  FrntSuspDamping=0.5  RearSuspDamping=0.5  FrntRollbarScaling=0.15  RearRollbarScaling=0.15  ABSEnable=off  TCSEnable=off  Cy_f=70e3  Cy_r=70e3  FrntSlipThreshold=0.2  RearSlipThreshold=0.2  FrntSkidThreshold=0.5  RearSkidThreshold=0.5  FrntSideSlipModifier=1  RearSideSlipModifier=1  ExtMu=off  lambda_mu=1.0  VehLightsControl=off  HeadlightColor=[ 1, 1, 1 ]  HighBeamIntensity=100000  LowBeamIntensity=60000  HighBeamConeAngle=1.22  LowBeamConeAngle=1.22  LeftHeadlightOrientation=[ 0, 0 ]  RightHeadlightOrientation=[ 0, 0 ]  BrakelightIntensity=500  ReverselightIntensity=500  SignallightIntensity=500  SignallightPeriod=1  SignalPulseWidth=50  StandardOutportEnabled=on  TransformOutportEnabled=off  SampleTime=-1  ActorType=SimulinkVehicle  ID=5  aMode=2  ActorTag=SimulinkVehicle5  CoordinateScheme=SAE
      settings: LibrarySourceBlock=vehdynlibsim3d/Simulation 3D Physics Vehicle
  CurrSpeed : Outport
  CurrVehicleInfo : Outport  Port=2  VectorParamsAs1DForOutWhenUnconnected=off
  Out1 : Outport  Port=3
  wires:
  DecelCmd/1 -> Simulation 3D Physics Vehicle2/3
  AccelCmd/1 -> Simulation 3D Physics Vehicle2/2
  SteerCmd/1 -> Delayed Steering System/1(SteerCmd)
  Gain/1 -> Pack Current States1/1(CurrSteer), Simulation 3D Physics Vehicle2/1
  Degrees to Radians1/1 -> Gain/1
  Delayed Steering System/1(CurrSteer) -> Degrees to Radians1/1
  Constant2/1 -> Pack Current States1/5(Direction), Simulation 3D Physics Vehicle2/4
  Simulation 3D Physics Vehicle2/5 -> Pack Current States1/4(CurrYawRate)
  Simulation 3D Physics Vehicle2/3 -> Matrix Concatenate/2, Calculate Norm1/1(Lateral Velocity)
  Simulation 3D Physics Vehicle2/1 -> Pack Current States1/2(Info)
  Simulation 3D Physics Vehicle2/2 -> Calculate Norm1/2(Longitudinal Velocity), Matrix Concatenate/1, Pack Current States1/3(CurrVelocity)
  Pack Current States1/1(CurrVehicleInfo) -> CurrVehicleInfo/1
  Calculate Norm1/1(Speed) -> CurrSpeed/1
  Constant/1 -> Matrix Concatenate/3
  Matrix Concatenate/1 -> Out1/1

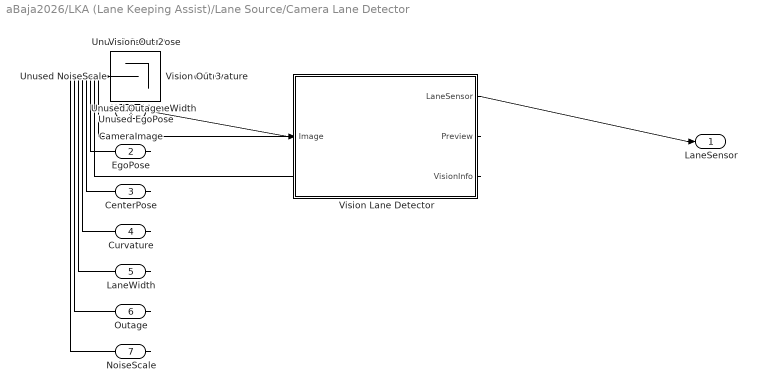
== system aBaja2026/LKA (Lane Keeping Assist)/Lane Source/Camera Lane Detector ==
  CameraImage : Inport
  EgoPose : Inport  Port=2
  CenterPose : Inport  Port=3
  Curvature : Inport  Port=4
  LaneWidth : Inport  Port=5
  Outage : Inport  Port=6
  NoiseScale : Inport  Port=7
  Unused CenterPose : Terminator
  Unused Curvature : Terminator
  Unused EgoPose : Terminator
  Unused LaneWidth : Terminator
  Unused NoiseScale : Terminator
  Unused Outage : Terminator
  Vision Lane Detector : Subsystem
  Vision Out 2 : Terminator
  Vision Out 3 : Terminator
  LaneSensor : Outport
  wires:
  CameraImage/1 -> Vision Lane Detector/1(Image)
  Vision Lane Detector/1(LaneSensor) -> LaneSensor/1
  Vision Lane Detector/2(Preview) -> Vision Out 2/1
  Vision Lane Detector/3(VisionInfo) -> Vision Out 3/1
  EgoPose/1 -> Unused EgoPose/1
  CenterPose/1 -> Unused CenterPose/1
  Curvature/1 -> Unused Curvature/1
  LaneWidth/1 -> Unused LaneWidth/1
  Outage/1 -> Unused Outage/1
  NoiseScale/1 -> Unused NoiseScale/1

== system aBaja2026/LKA (Lane Keeping Assist)/Lane Source/Emulated Lane Sensor (development only) ==
  CameraImage : Inport
  EgoPose : Inport  Port=2
  CenterPose : Inport  Port=3
  Curvature : Inport  Port=4
  LaneWidth : Inport  Port=5
  Outage : Inport  Port=6
  NoiseScale : Inport  Port=7
  Unused CameraImage : Terminator
  Virtual Lane Sensor : Subsystem  ReferencedSubsystem=VirtualLaneSensor
  LaneSensor : Outport
  wires:
  EgoPose/1 -> Virtual Lane Sensor/1
  CenterPose/1 -> Virtual Lane Sensor/2
  Curvature/1 -> Virtual Lane Sensor/3
  LaneWidth/1 -> Virtual Lane Sensor/4
  Outage/1 -> Virtual Lane Sensor/5
  NoiseScale/1 -> Virtual Lane Sensor/6
  Virtual Lane Sensor/1 -> LaneSensor/1
  CameraImage/1 -> Unused CameraImage/1

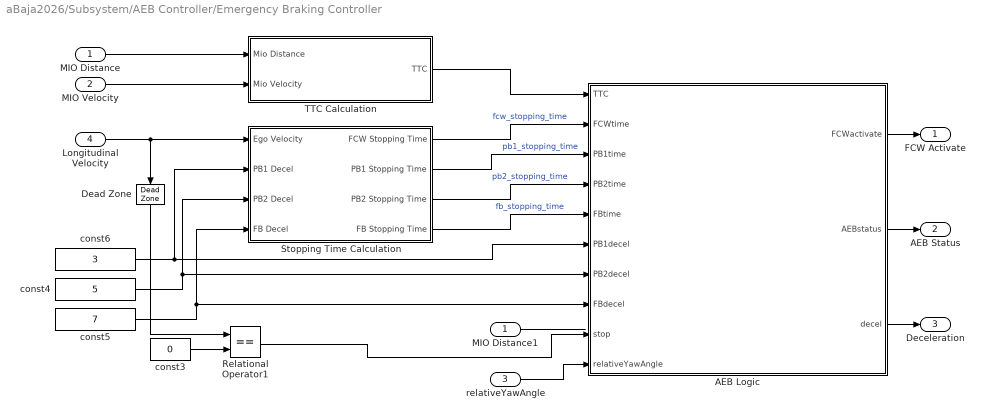
== system aBaja2026/Subsystem/AEB Controller/Emergency Braking Controller ==
  MIO Distance : Inport
  MIO Velocity : Inport  Port=2
  relativeYawAngle : Inport  Port=3
  Longitudinal Velocity : Inport  Port=4
  AEB Logic : Stateflow chart  TreatAsAtomicUnit=on
  Dead Zone : DeadZone  LowerValue=-inf  UpperValue=0.001
  MIO Distance1 : InportShadow
  Relational Operator1 : RelationalOperator  Operator===  OutDataTypeStr=boolean  RndMeth=Simplest  InputSameDT=off
  Stopping Time Calculation : Subsystem
  TTC Calculation : Subsystem
  const3 : Constant  Value=0  SampleTime=-1
  const4 : Constant  Value=5  SampleTime=-1
  const5 : Constant  Value=7  SampleTime=-1
  const6 : Constant  Value=3  SampleTime=-1
  FCW Activate : Outport  VectorParamsAs1DForOutWhenUnconnected=off
  AEB Status : Outport  Port=2  VectorParamsAs1DForOutWhenUnconnected=off
  Deceleration : Outport  Port=3  OutDataTypeStr=double  VectorParamsAs1DForOutWhenUnconnected=off
  wires:
  AEB Logic/3(decel) -> Deceleration/1
  const4/1 -> AEB Logic/7(PB2decel), Stopping Time Calculation/3(PB2 Decel)
  const5/1 -> Stopping Time Calculation/4(FB Decel), AEB Logic/8(FBdecel)
  AEB Logic/2(AEBstatus) -> AEB Status/1
  const3/1 -> Relational Operator1/2
  const6/1 -> AEB Logic/6(PB1decel), Stopping Time Calculation/2(PB1 Decel)
  Stopping Time Calculation/3(PB2 Stopping Time) -> AEB Logic/4(PB2time)  "pb2_stopping_time"
  Stopping Time Calculation/2(PB1 Stopping Time) -> AEB Logic/3(PB1time)  "pb1_stopping_time"
  Stopping Time Calculation/4(FB Stopping Time) -> AEB Logic/5(FBtime)  "fb_stopping_time"
  Stopping Time Calculation/1(FCW Stopping Time) -> AEB Logic/2(FCWtime)  "fcw_stopping_time"
  AEB Logic/1(FCWactivate) -> FCW Activate/1
  MIO Distance/1 -> TTC Calculation/1(Mio Distance)
  MIO Velocity/1 -> TTC Calculation/2(Mio Velocity)
  TTC Calculation/1(TTC) -> AEB Logic/1(TTC)
  Longitudinal Velocity/1 -> Dead Zone/1, Stopping Time Calculation/1(Ego Velocity)
  Relational Operator1/1 -> AEB Logic/9(stop)
  MIO Distance1/1 -> ?
  relativeYawAngle/1 -> AEB Logic/10(relativeYawAngle)
  Dead Zone/1 -> Relational Operator1/1

== system aBaja2026/Subsystem2/Initialize State/Calculate Initial States ==
  EgoRuntime : Inport
  Trigger : TriggerPort  VariantControl=(inherit)  InitialTriggerSignalState=negative  PortDimensions=1
  Calculate Initial States : MATLAB Function  TreatAsAtomicUnit=on
  EgoInitialState : Outport
  wires:
  EgoRuntime/1 -> Calculate Initial States/1(egoRuntime)
  Calculate Initial States/1(egoInitialState) -> EgoInitialState/1

== system aBaja2026/Subsystem2/Subsystem1/Switch Case Action Subsystem ==
  Driver_SteerCmd : Inport
  Controller_AccelCmd : Inport  Port=2
  Controller_DecelCmd : Inport  Port=3
  Action Port : ActionPort  ActionPortLabel=case [ 0 ]:
  Steer : Outport
  Accel : Outport  Port=2
  Decel : Outport  Port=3
  wires:
  Driver_SteerCmd/1 -> Steer/1
  Controller_AccelCmd/1 -> Accel/1
  Controller_DecelCmd/1 -> Decel/1

== system aBaja2026/Subsystem2/Subsystem1/Switch Case Action Subsystem1 ==
  Driver_AccelCmd : Inport
  Driver_DecelCmd : Inport  Port=2
  Controller_SteerCmd : Inport  Port=3
  Action Port : ActionPort  ActionPortLabel=case [ 1 ]:
  Steer : Outport
  Accel : Outport  Port=2
  Decel : Outport  Port=3
  wires:
  Driver_AccelCmd/1 -> Accel/1
  Driver_DecelCmd/1 -> Decel/1
  Controller_SteerCmd/1 -> Steer/1

== system aBaja2026/Subsystem2/Subsystem1/Switch Case Action Subsystem2 ==
  Controller_SteerCmd : Inport
  Controller_AccelCmd : Inport  Port=2
  Controller_DecelCmd : Inport  Port=3
  Action Port : ActionPort  ActionPortLabel=case [ 2 ]:
  Steer : Outport
  Accel : Outport  Port=2
  Decel : Outport  Port=3
  wires:
  Controller_SteerCmd/1 -> Steer/1
  Controller_AccelCmd/1 -> Accel/1
  Controller_DecelCmd/1 -> Decel/1

== system aBaja2026/Subsystem2/Subsystem1/Switch Case Action Subsystem3 ==
  Driver_SteerCmd : Inport
  Driver_AccelCmd : Inport  Port=2
  Driver_DecelCmd : Inport  Port=3
  Action Port : ActionPort  ActionPortLabel=case [ 3 ]:
  Steer : Outport
  Accel : Outport  Port=2
  Decel : Outport  Port=3
  wires:
  Driver_SteerCmd/1 -> Steer/1
  Driver_AccelCmd/1 -> Accel/1
  Driver_DecelCmd/1 -> Decel/1

== system aBaja2026/Subsystem2/Vehicle Dynamics/Calculate Norm1 ==
  Lateral Velocity : Inport
  Longitudinal Velocity : Inport  Port=2
  Add : Sum
  Math Function : Math  Operator=square
  Math Function1 : Math  Operator=square
  Sqrt : Sqrt
  Speed : Outport
  wires:
  Longitudinal Velocity/1 -> Math Function1/1
  Lateral Velocity/1 -> Math Function/1
  Sqrt/1 -> Speed/1
  Math Function/1 -> Add/1
  Math Function1/1 -> Add/2
  Add/1 -> Sqrt/1

== system aBaja2026/Subsystem2/Vehicle Dynamics/Delayed Steering System ==
  SteerCmd : Inport
  Add : Sum  Inputs=+-
  Delay : TransferFcn  Denominator=[0.1 0]
  CurrSteer : Outport  VectorParamsAs1DForOutWhenUnconnected=off
  wires:
  Add/1 -> Delay/1
  SteerCmd/1 -> Add/1
  Delay/1 -> CurrSteer/1, Add/2

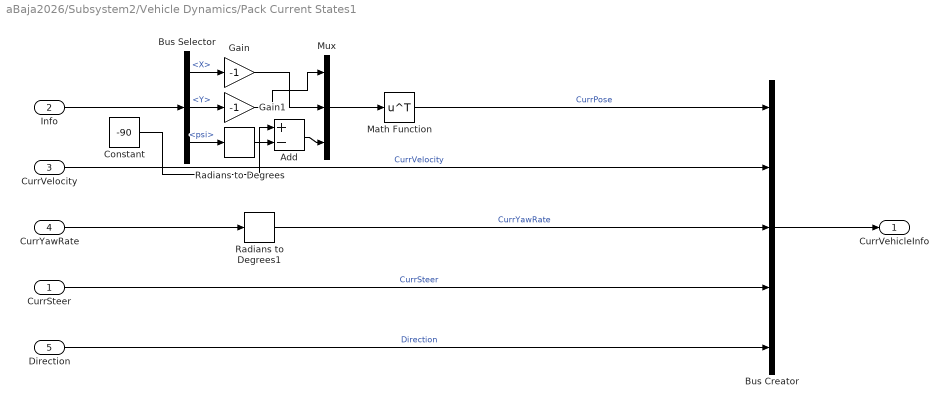
== system aBaja2026/Subsystem2/Vehicle Dynamics/Pack Current States1 ==
  CurrSteer : Inport
  Info : Inport  Port=2
  CurrVelocity : Inport  Port=3
  CurrYawRate : Inport  Port=4
  Direction : Inport  Port=5
  Add : Sum  Inputs=+-
  Bus Creator : BusCreator  Inputs=5  OutDataTypeStr=Bus: BusVehicleInfo  NonVirtualBus=on
      settings: InheritFromInputs=off
  Bus Selector : BusSelector  OutputSignals=InertFrm.Cg.Disp.X,InertFrm.Cg.Disp.Y,InertFrm.Cg.Ang.psi
  Constant : Constant  Value=-90
  Gain : Gain  Gain=-1
  Gain1 : Gain  Gain=-1
  Math Function : Math  Operator=transpose  SignedPower=on
  Mux : Mux  Inputs=3
  Radians to Degrees : simulink_extras/Transformations/Radians to Degrees
  Radians to Degrees1 : simulink_extras/Transformations/Radians to Degrees
  CurrVehicleInfo : Outport  VectorParamsAs1DForOutWhenUnconnected=off
  wires:
  Radians to Degrees1/1 -> Bus Creator/3  "CurrYawRate"
  Bus Creator/1 -> CurrVehicleInfo/1
  Info/1 -> Bus Selector/1
  Mux/1 -> Math Function/1
  Direction/1 -> Bus Creator/5  "Direction"
  CurrYawRate/1 -> Radians to Degrees1/1
  Math Function/1 -> Bus Creator/1  "CurrPose"
  CurrSteer/1 -> Bus Creator/4  "CurrSteer"
  CurrVelocity/1 -> Bus Creator/2  "CurrVelocity"
  Bus Selector/3 -> Radians to Degrees/1  "<psi>"
  Bus Selector/1 -> Gain/1  "<X>"
  Bus Selector/2 -> Gain1/1  "<Y>"
  Gain/1 -> Mux/2
  Gain1/1 -> Mux/1
  Radians to Degrees/1 -> Add/2
  Add/1 -> Mux/3
  Constant/1 -> Add/1
